simulink model "Q3_Uniform"  (R2024b)
settings: Solver=FixedStepDiscrete  StartTime=0.0  StopTime=1  RelTol=1e-3
libraries: spsControlledVoltageSourceLib x1, spsCurrentMeasurementLib x1, spsGroundLib x1, spsPVArrayLib x1, simulink x1, spsVoltageMeasurementLib x1, sps_lib x1
settings Model: Creator=mehme  LastModifiedBy=mehme

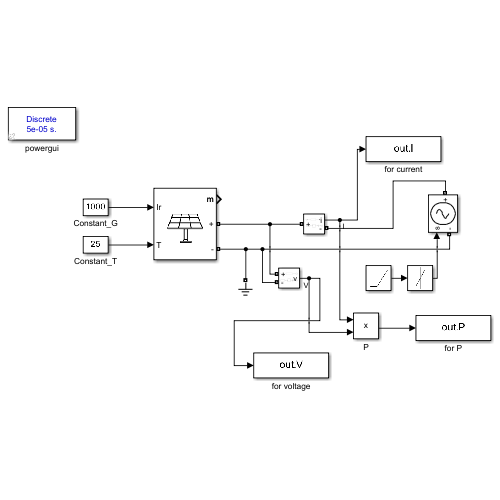
[thumbnail: Simulink's stored preview of the top-level diagram]
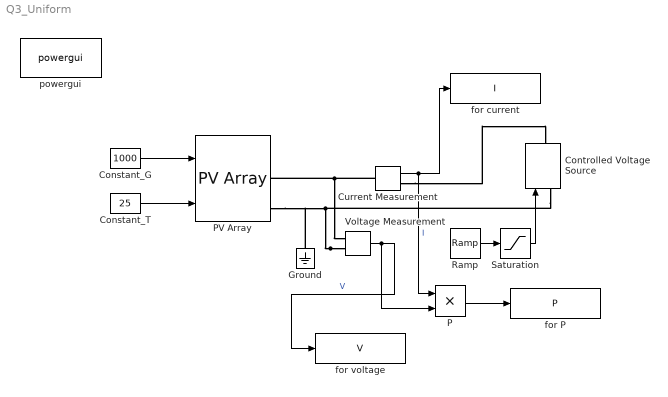
== system Q3_Uniform ==
  Constant_G : Constant  Value=1000
  Constant_T : Constant  Value=25
  Controlled Voltage Source : spsControlledVoltageSourceLib/Controlled Voltage Source  Initialize=on  Source_Type=AC  Amplitude=0  Phase=0  Frequency=0  Measurements=None
  Current Measurement : spsCurrentMeasurementLib/Current Measurement  PhasorSimulation=off  OutputType=Complex  PSBequivalent=0
  Ground : spsGroundLib/Ground  LConnTagsString=a
  P : Product
  PV Array : spsPVArrayLib/PV Array  Npar=7  Nser=18  PlotType=array @ 1000 W/m2 & specified temperatures  S_vec="[ 1000  500  100 ]"  Temp_C_vec=[25]  ModuleName=User-defined  PlotWhenSelected=off  Pm=415.168  Ncell=72  Voc=49.6  Isc=10.86  Vm=41.6  Im=9.98  beta_Voc_pc=-0.36099  alpha_Isc_pc=0.102  beta_Voc=-0.17905  alpha_Isc=0.011077  IL=10.8339  I0=4.0048e-10  nI=1.1179  Rsh=129.3253  Rs=0.17235  RobustModel=off  RobustCellTemperature=313.3991  BAL=on  Tc=1e-6  Tfilter=5e-5
  Ramp : simulink/Sources/Ramp  slope=900  start=0  InitialOutput=0
  Saturation : Saturate  UpperLimit=900  LowerLimit=0
  Voltage Measurement : spsVoltageMeasurementLib/Voltage Measurement  PhasorSimulation=off  OutputType=Complex  PSBequivalent=0
  for P : ToWorkspace  VariableName=P  SampleTime=-1
  for current : ToWorkspace  VariableName=I  SampleTime=-1
  for voltage : ToWorkspace  VariableName=V  SampleTime=-1
  powergui : sps_lib/powergui  Priority=1  SimulationMode=Discrete  SampleTime=5e-5  frequency=60  Iterations=50  frequencyindice=0  Pbase=100e6  ErrMax=1e-4  UnitsV=kV  UnitsW=MW  buscounter=0  FunctionMessages=off  echomessages=off  EnableUseOfTLC=off  CurrentSourceSwitches=off  DisableSnubberDevices=off  DisableRonSwitches=off  DisableVfSwitches=off  DisplayEquations=off  AutomaticDiscreteSolvers=off  SolverType=Tustin/Backward Euler (TBE)  Interpol=off  ExternalGateDelay=off  methode=off  Ts=100  x0status=blocks  SPID=on  SwTol=0  HookPort=off  NonlinearTolerance=1e-4  nMaxIteration=100  ContinueOnMaxIteration=off  RestoreLinks=warning  ResistiveCurrentMeasurement=off  Frange=[0:2:500]  Ylog=off  Xlog=on  ShowGrid=off  save=off  variable=ZData  structure=0  ZoomFFT=off  StartTime=0.0  cycles=1  DisplayStyle=1  fundamental=60  FreqAxis=off  MaxFrequency=1000  frequencyindicesteady=1  RmsSteady=1  display=off
  wires:
  Voltage Measurement/1 -> P/2, for voltage/1  "V"
  Current Measurement/1 -> for current/1, P/1  "I"
  P/1 -> for P/1
  Ramp/1 -> Saturation/1
  Saturation/1 -> Controlled Voltage Source/1
  Constant_G/1 -> PV Array/1
  Constant_T/1 -> PV Array/2
  connections:
  Current Measurement/LConn1 -- Voltage Measurement/LConn1 -- PV Array/RConn1
  Current Measurement/RConn1 -- Controlled Voltage Source/RConn1
  Voltage Measurement/LConn2 -- Ground/LConn1 -- PV Array/RConn2 -- Controlled Voltage Source/LConn1
